simulink model "FSI07"  (R2024b)
settings: Solver=VariableStepAuto  StartTime=0.0  StopTime=t_stop  FixedStep=0.001  MaxStep=0.001  RelTol=1e-3
values from neighbouring files (symbols this model uses):
  cphi = 0.1    [FSI05WS.m]    (also in FSI06WS.m; FSI07WS.m)
  I0 = 0    [FSI03WS.m]    (also in FSI05WS.m = 0.0001; FSI06WS.m = 0.0001; FSI07WS.m = 0.0001)
  I_regulator_D = 0    [FSI07WS.m]
  I_regulator_I = 100000    [FSI07WS.m]
  I_regulator_N = 0    [FSI07WS.m]
  I_regulator_P = 1000    [FSI07WS.m]
  I_zadana = 0    [FSI07WS.m]
  integrator = 10    [FSI07WS.m]
  L = 0.02    [FSI03WS.m]    (also in FSI05WS.m = 0.05; FSI06WS.m = 0.05; FSI07WS.m = 0.05; FSI10WS.m = 0.3)
  M = 0    [FSI05WS.m]    (also in FSI06WS.m = 0.2; FSI07WS.m = 0.04; FSI10WS.m = 3)
  omega_zadana = 100    [FSI06WS.m]    (also in FSI07WS.m)
  R = 5    [FSI03WS.m]    (also in FSI05WS.m = 0; FSI06WS.m = 20; FSI07WS.m = 20)
  saturator = 0.5    [FSI07WS.m]
  step_t = 2    [FSI05WS.m]    (also in FSI06WS.m = 1; FSI07WS.m = 0.5)
  w_regulator_D = 0    [FSI07WS.m]
  w_regulator_I = 100    [FSI07WS.m]
  w_regulator_N = 0    [FSI07WS.m]
  w_regulator_P = 4    [FSI07WS.m]
libraries: slpidlib x4
settings Model: Creator=fmiro  LastModifiedBy=fmiro

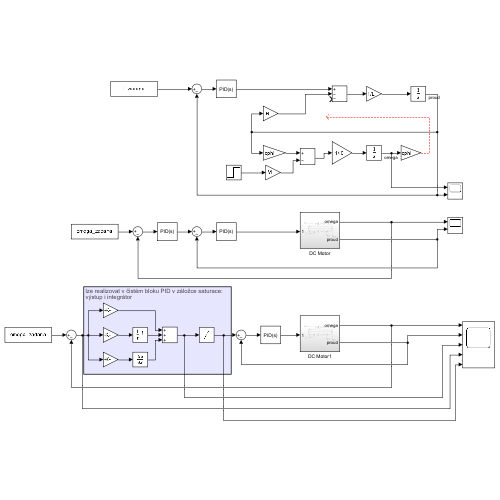
[thumbnail: Simulink's stored preview of the top-level diagram]
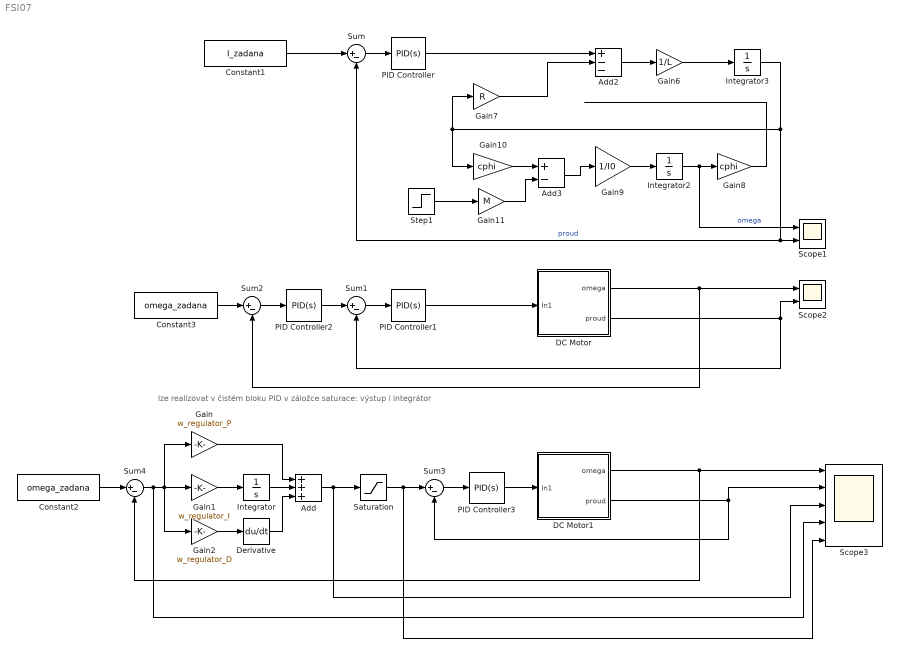
== system FSI07 ==
  note: lze realizovat v čistém bloku PID v záložce saturace:
      | výstup i integrátor
  Add : Sum  Inputs=+++
  Add2 : Sum  Inputs=+--
  Add3 : Sum  Inputs=+-
  Constant1 : Constant  Value=I_zadana
  Constant2 : Constant  Value=omega_zadana
  Constant3 : Constant  Value=omega_zadana
  DC Motor : Subsystem
  DC Motor1 : Subsystem
  Derivative : Derivative
  Gain : Gain  Gain=w_regulator_P
  Gain1 : Gain  Gain=w_regulator_I
  Gain10 : Gain  Gain=cphi
  Gain11 : Gain  Gain=M
  Gain2 : Gain  Gain=w_regulator_D
  Gain6 : Gain  Gain=1/L
  Gain7 : Gain  Gain=R
  Gain8 : Gain  Gain=cphi
  Gain9 : Gain  Gain=1/I0
  Integrator : Integrator  LimitOutput=on  UpperSaturationLimit=integrator  LowerSaturationLimit=-integrator
  Integrator2 : Integrator
  Integrator3 : Integrator
  PID Controller : slpidlib/PID Controller  Controller=PID  Form=Parallel  TimeDomain=Continuous-time  UseExternalTs=off  SampleTime=-1  IntegratorMethod=Forward Euler  FilterMethod=Forward Euler  ControllerParametersSource=internal  P=I_regulator_P  I=I_regulator_I  UseKiTs=off  D=I_regulator_D  UseExternalDerivativeSource=off  N=I_regulator_N  UseFilter=on  TunerSelectOption=Transfer Function Based (PID Tuner App)  InitialConditionSource=internal  InitialConditionForIntegrator=0  InitialConditionForFilter=0  DifferentiatorICPrevScaledInput=0  ExternalReset=none  TrackingMode=off  Kt=1  LimitOutput=off  SatLimitsSource=internal  UpperSaturationLimit=inf  LowerSaturationLimit=-inf  LinearizeAsGain=on  AntiWindupMode=none  Kb=1  LimitIntegrator=off  UpperIntegratorSaturationLimit=inf  LowerIntegratorSaturationLimit=-inf  POutMin=[]  POutMax=[]  IOutMin=[]  IOutMax=[]  DOutMin=[]  DOutMax=[]  NOutMin=[]  NOutMax=[]  SumOutMin=[]  SumOutMax=[]  SaturationOutMin=[]  SaturationOutMax=[]  PParamMin=[]  PParamMax=[]  IParamMin=[]  IParamMax=[]  DParamMin=[]  DParamMax=[]  NParamMin=[]  NParamMax=[]  KbParamMin=[]  KbParamMax=[]  KtParamMin=[]  KtParamMax=[]  KbOutMin=[]  KbOutMax=[]  KtOutMin=[]  KtOutMax=[]  IntegratorOutMin=[]  IntegratorOutMax=[]  FilterOutMin=[]  FilterOutMax=[]  SumI1OutMin=[]  SumI1OutMax=[]  SumI2OutMin=[]  SumI2OutMax=[]  SumI3OutMin=[]  SumI3OutMax=[]  SumI4OutMin=[]  SumI4OutMax=[]  SumDOutMin=[]  SumDOutMax=[]  DifferentiatorOutMin=[]  DifferentiatorOutMax=[]  FilterDiffOutCoefMin=[]  FilterDiffOutCoefMax=[]  ReciprocalOutMin=[]  ReciprocalOutMax=[]  SumDenOutMin=[]  SumDenOutMax=[]  SumNumOutMin=[]  SumNumOutMax=[]  DivideOutMin=[]  DivideOutMax=[]  UdiffTsProdOutMin=[]  UdiffTsProdOutMax=[]  NTsProdOutMin=[]  NTsProdOutMax=[]  UintegralTsProdOutMin=[]  UintegralTsProdOutMax=[]  UngainTsProdOutMin=[]  UngainTsProdOutMax=[]  ClampingZeroOutDataTypeStr=Inherit: Inherit via back propagation  ClampingZeroOutMin=[]  ClampingZeroOutMax=[]  FilterDenConstantOutDataTypeStr=Inherit: Inherit via back propagation  FilterDenConstantOutMin=[]  FilterDenConstantOutMax=[]  PCopyOutDataTypeStr=Inherit: Inherit via back propagation  PCopyOutMin=[]  PCopyOutMax=[]  NCopyOutDataTypeStr=Inherit: Inherit via back propagation  NCopyOutMin=[]  NCopyOutMax=[]  IntegratorContinuousStateAttributes=''  IntegratorStateMustResolveToSignalObject=off  IntegratorRTWStateStorageClass=Auto  FilterContinuousStateAttributes=''  FilterStateMustResolveToSignalObject=off  FilterRTWStateStorageClass=Auto  ParallelPVariant=InternalParameters  IdealPVariant=Disabled  IVariant=InternalParameters  DVariant=InternalParameters  IntegratorVariant=Continuous  SatVariant=Disabled  AWVariant=Passthrough  PCopyVariant=Disabled  TRVariant=Disabled  FdbkBlocksVariant=Forward  IdealPFdbkVariant=Disabled  SatFdbkVariant=Disabled  DerivativeFilterVariant=ContFilter  NVariant=InternalParameters  NCopyVariant=Disabled  FilterICVariant=InternalICsFilter  IntegratorICVariant=InternalICs  ExternalResetVariant=Disabled  TRSumVariant=Passthrough  SumFdbkVariant=Disabled  SumVariant=Sum_PID  TsampFilterVariant=InternalTs  TsampNgainVariant=Passthrough  TsampIntegralVariant=Disabled_SignalSpec  ExternalSaturationOutDataTypeStr=Inherit: Same as second input  DerivativeSourceVariant=ErrorSignal  PreIntVariant=InternalPreInt
  PID Controller1 : slpidlib/PID Controller  Controller=PID  Form=Parallel  TimeDomain=Continuous-time  UseExternalTs=off  SampleTime=-1  IntegratorMethod=Forward Euler  FilterMethod=Forward Euler  ControllerParametersSource=internal  P=I_regulator_P  I=I_regulator_I  UseKiTs=off  D=I_regulator_D  UseExternalDerivativeSource=off  N=I_regulator_N  UseFilter=on  TunerSelectOption=Transfer Function Based (PID Tuner App)  InitialConditionSource=internal  InitialConditionForIntegrator=0  InitialConditionForFilter=0  DifferentiatorICPrevScaledInput=0  ExternalReset=none  TrackingMode=off  Kt=1  LimitOutput=off  SatLimitsSource=internal  UpperSaturationLimit=inf  LowerSaturationLimit=-inf  LinearizeAsGain=on  AntiWindupMode=none  Kb=1  LimitIntegrator=off  UpperIntegratorSaturationLimit=inf  LowerIntegratorSaturationLimit=-inf  POutMin=[]  POutMax=[]  IOutMin=[]  IOutMax=[]  DOutMin=[]  DOutMax=[]  NOutMin=[]  NOutMax=[]  SumOutMin=[]  SumOutMax=[]  SaturationOutMin=[]  SaturationOutMax=[]  PParamMin=[]  PParamMax=[]  IParamMin=[]  IParamMax=[]  DParamMin=[]  DParamMax=[]  NParamMin=[]  NParamMax=[]  KbParamMin=[]  KbParamMax=[]  KtParamMin=[]  KtParamMax=[]  KbOutMin=[]  KbOutMax=[]  KtOutMin=[]  KtOutMax=[]  IntegratorOutMin=[]  IntegratorOutMax=[]  FilterOutMin=[]  FilterOutMax=[]  SumI1OutMin=[]  SumI1OutMax=[]  SumI2OutMin=[]  SumI2OutMax=[]  SumI3OutMin=[]  SumI3OutMax=[]  SumI4OutMin=[]  SumI4OutMax=[]  SumDOutMin=[]  SumDOutMax=[]  DifferentiatorOutMin=[]  DifferentiatorOutMax=[]  FilterDiffOutCoefMin=[]  FilterDiffOutCoefMax=[]  ReciprocalOutMin=[]  ReciprocalOutMax=[]  SumDenOutMin=[]  SumDenOutMax=[]  SumNumOutMin=[]  SumNumOutMax=[]  DivideOutMin=[]  DivideOutMax=[]  UdiffTsProdOutMin=[]  UdiffTsProdOutMax=[]  NTsProdOutMin=[]  NTsProdOutMax=[]  UintegralTsProdOutMin=[]  UintegralTsProdOutMax=[]  UngainTsProdOutMin=[]  UngainTsProdOutMax=[]  ClampingZeroOutDataTypeStr=Inherit: Inherit via back propagation  ClampingZeroOutMin=[]  ClampingZeroOutMax=[]  FilterDenConstantOutDataTypeStr=Inherit: Inherit via back propagation  FilterDenConstantOutMin=[]  FilterDenConstantOutMax=[]  PCopyOutDataTypeStr=Inherit: Inherit via back propagation  PCopyOutMin=[]  PCopyOutMax=[]  NCopyOutDataTypeStr=Inherit: Inherit via back propagation  NCopyOutMin=[]  NCopyOutMax=[]  IntegratorContinuousStateAttributes=''  IntegratorStateMustResolveToSignalObject=off  IntegratorRTWStateStorageClass=Auto  FilterContinuousStateAttributes=''  FilterStateMustResolveToSignalObject=off  FilterRTWStateStorageClass=Auto  ParallelPVariant=InternalParameters  IdealPVariant=Disabled  IVariant=InternalParameters  DVariant=InternalParameters  IntegratorVariant=Continuous  SatVariant=Disabled  AWVariant=Passthrough  PCopyVariant=Disabled  TRVariant=Disabled  FdbkBlocksVariant=Forward  IdealPFdbkVariant=Disabled  SatFdbkVariant=Disabled  DerivativeFilterVariant=ContFilter  NVariant=InternalParameters  NCopyVariant=Disabled  FilterICVariant=InternalICsFilter  IntegratorICVariant=InternalICs  ExternalResetVariant=Disabled  TRSumVariant=Passthrough  SumFdbkVariant=Disabled  SumVariant=Sum_PID  TsampFilterVariant=InternalTs  TsampNgainVariant=Passthrough  TsampIntegralVariant=Disabled_SignalSpec  ExternalSaturationOutDataTypeStr=Inherit: Same as second input  DerivativeSourceVariant=ErrorSignal  PreIntVariant=InternalPreInt
  PID Controller2 : slpidlib/PID Controller  Controller=PID  Form=Parallel  TimeDomain=Continuous-time  UseExternalTs=off  SampleTime=-1  IntegratorMethod=Forward Euler  FilterMethod=Forward Euler  ControllerParametersSource=internal  P=w_regulator_P  I=w_regulator_I  UseKiTs=off  D=w_regulator_D  UseExternalDerivativeSource=off  N=w_regulator_N  UseFilter=on  TunerSelectOption=Transfer Function Based (PID Tuner App)  InitialConditionSource=internal  InitialConditionForIntegrator=0  InitialConditionForFilter=0  DifferentiatorICPrevScaledInput=0  ExternalReset=none  TrackingMode=off  Kt=1  LimitOutput=off  SatLimitsSource=internal  UpperSaturationLimit=inf  LowerSaturationLimit=-inf  LinearizeAsGain=on  AntiWindupMode=none  Kb=1  LimitIntegrator=off  UpperIntegratorSaturationLimit=inf  LowerIntegratorSaturationLimit=-inf  POutMin=[]  POutMax=[]  IOutMin=[]  IOutMax=[]  DOutMin=[]  DOutMax=[]  NOutMin=[]  NOutMax=[]  SumOutMin=[]  SumOutMax=[]  SaturationOutMin=[]  SaturationOutMax=[]  PParamMin=[]  PParamMax=[]  IParamMin=[]  IParamMax=[]  DParamMin=[]  DParamMax=[]  NParamMin=[]  NParamMax=[]  KbParamMin=[]  KbParamMax=[]  KtParamMin=[]  KtParamMax=[]  KbOutMin=[]  KbOutMax=[]  KtOutMin=[]  KtOutMax=[]  IntegratorOutMin=[]  IntegratorOutMax=[]  FilterOutMin=[]  FilterOutMax=[]  SumI1OutMin=[]  SumI1OutMax=[]  SumI2OutMin=[]  SumI2OutMax=[]  SumI3OutMin=[]  SumI3OutMax=[]  SumI4OutMin=[]  SumI4OutMax=[]  SumDOutMin=[]  SumDOutMax=[]  DifferentiatorOutMin=[]  DifferentiatorOutMax=[]  FilterDiffOutCoefMin=[]  FilterDiffOutCoefMax=[]  ReciprocalOutMin=[]  ReciprocalOutMax=[]  SumDenOutMin=[]  SumDenOutMax=[]  SumNumOutMin=[]  SumNumOutMax=[]  DivideOutMin=[]  DivideOutMax=[]  UdiffTsProdOutMin=[]  UdiffTsProdOutMax=[]  NTsProdOutMin=[]  NTsProdOutMax=[]  UintegralTsProdOutMin=[]  UintegralTsProdOutMax=[]  UngainTsProdOutMin=[]  UngainTsProdOutMax=[]  ClampingZeroOutDataTypeStr=Inherit: Inherit via back propagation  ClampingZeroOutMin=[]  ClampingZeroOutMax=[]  FilterDenConstantOutDataTypeStr=Inherit: Inherit via back propagation  FilterDenConstantOutMin=[]  FilterDenConstantOutMax=[]  PCopyOutDataTypeStr=Inherit: Inherit via back propagation  PCopyOutMin=[]  PCopyOutMax=[]  NCopyOutDataTypeStr=Inherit: Inherit via back propagation  NCopyOutMin=[]  NCopyOutMax=[]  IntegratorContinuousStateAttributes=''  IntegratorStateMustResolveToSignalObject=off  IntegratorRTWStateStorageClass=Auto  FilterContinuousStateAttributes=''  FilterStateMustResolveToSignalObject=off  FilterRTWStateStorageClass=Auto  ParallelPVariant=InternalParameters  IdealPVariant=Disabled  IVariant=InternalParameters  DVariant=InternalParameters  IntegratorVariant=Continuous  SatVariant=Disabled  AWVariant=Passthrough  PCopyVariant=Disabled  TRVariant=Disabled  FdbkBlocksVariant=Forward  IdealPFdbkVariant=Disabled  SatFdbkVariant=Disabled  DerivativeFilterVariant=ContFilter  NVariant=InternalParameters  NCopyVariant=Disabled  FilterICVariant=InternalICsFilter  IntegratorICVariant=InternalICs  ExternalResetVariant=Disabled  TRSumVariant=Passthrough  SumFdbkVariant=Disabled  SumVariant=Sum_PID  TsampFilterVariant=InternalTs  TsampNgainVariant=Passthrough  TsampIntegralVariant=Disabled_SignalSpec  ExternalSaturationOutDataTypeStr=Inherit: Same as second input  DerivativeSourceVariant=ErrorSignal  PreIntVariant=InternalPreInt
  PID Controller3 : slpidlib/PID Controller  Controller=PID  Form=Parallel  TimeDomain=Continuous-time  UseExternalTs=off  SampleTime=-1  IntegratorMethod=Forward Euler  FilterMethod=Forward Euler  ControllerParametersSource=internal  P=I_regulator_P  I=I_regulator_I  UseKiTs=off  D=I_regulator_D  UseExternalDerivativeSource=off  N=I_regulator_N  UseFilter=on  TunerSelectOption=Transfer Function Based (PID Tuner App)  InitialConditionSource=internal  InitialConditionForIntegrator=0  InitialConditionForFilter=0  DifferentiatorICPrevScaledInput=0  ExternalReset=none  TrackingMode=off  Kt=1  LimitOutput=off  SatLimitsSource=internal  UpperSaturationLimit=inf  LowerSaturationLimit=-inf  LinearizeAsGain=on  AntiWindupMode=none  Kb=1  LimitIntegrator=off  UpperIntegratorSaturationLimit=inf  LowerIntegratorSaturationLimit=-inf  POutMin=[]  POutMax=[]  IOutMin=[]  IOutMax=[]  DOutMin=[]  DOutMax=[]  NOutMin=[]  NOutMax=[]  SumOutMin=[]  SumOutMax=[]  SaturationOutMin=[]  SaturationOutMax=[]  PParamMin=[]  PParamMax=[]  IParamMin=[]  IParamMax=[]  DParamMin=[]  DParamMax=[]  NParamMin=[]  NParamMax=[]  KbParamMin=[]  KbParamMax=[]  KtParamMin=[]  KtParamMax=[]  KbOutMin=[]  KbOutMax=[]  KtOutMin=[]  KtOutMax=[]  IntegratorOutMin=[]  IntegratorOutMax=[]  FilterOutMin=[]  FilterOutMax=[]  SumI1OutMin=[]  SumI1OutMax=[]  SumI2OutMin=[]  SumI2OutMax=[]  SumI3OutMin=[]  SumI3OutMax=[]  SumI4OutMin=[]  SumI4OutMax=[]  SumDOutMin=[]  SumDOutMax=[]  DifferentiatorOutMin=[]  DifferentiatorOutMax=[]  FilterDiffOutCoefMin=[]  FilterDiffOutCoefMax=[]  ReciprocalOutMin=[]  ReciprocalOutMax=[]  SumDenOutMin=[]  SumDenOutMax=[]  SumNumOutMin=[]  SumNumOutMax=[]  DivideOutMin=[]  DivideOutMax=[]  UdiffTsProdOutMin=[]  UdiffTsProdOutMax=[]  NTsProdOutMin=[]  NTsProdOutMax=[]  UintegralTsProdOutMin=[]  UintegralTsProdOutMax=[]  UngainTsProdOutMin=[]  UngainTsProdOutMax=[]  ClampingZeroOutDataTypeStr=Inherit: Inherit via back propagation  ClampingZeroOutMin=[]  ClampingZeroOutMax=[]  FilterDenConstantOutDataTypeStr=Inherit: Inherit via back propagation  FilterDenConstantOutMin=[]  FilterDenConstantOutMax=[]  PCopyOutDataTypeStr=Inherit: Inherit via back propagation  PCopyOutMin=[]  PCopyOutMax=[]  NCopyOutDataTypeStr=Inherit: Inherit via back propagation  NCopyOutMin=[]  NCopyOutMax=[]  IntegratorContinuousStateAttributes=''  IntegratorStateMustResolveToSignalObject=off  IntegratorRTWStateStorageClass=Auto  FilterContinuousStateAttributes=''  FilterStateMustResolveToSignalObject=off  FilterRTWStateStorageClass=Auto  ParallelPVariant=InternalParameters  IdealPVariant=Disabled  IVariant=InternalParameters  DVariant=InternalParameters  IntegratorVariant=Continuous  SatVariant=Disabled  AWVariant=Passthrough  PCopyVariant=Disabled  TRVariant=Disabled  FdbkBlocksVariant=Forward  IdealPFdbkVariant=Disabled  SatFdbkVariant=Disabled  DerivativeFilterVariant=ContFilter  NVariant=InternalParameters  NCopyVariant=Disabled  FilterICVariant=InternalICsFilter  IntegratorICVariant=InternalICs  ExternalResetVariant=Disabled  TRSumVariant=Passthrough  SumFdbkVariant=Disabled  SumVariant=Sum_PID  TsampFilterVariant=InternalTs  TsampNgainVariant=Passthrough  TsampIntegralVariant=Disabled_SignalSpec  ExternalSaturationOutDataTypeStr=Inherit: Same as second input  DerivativeSourceVariant=ErrorSignal  PreIntVariant=InternalPreInt
  Saturation : Saturate  UpperLimit=saturator  LowerLimit=-saturator
  Scope1 : Scope  NumInputPorts=2
  Scope2 : Scope  NumInputPorts=2
  Scope3 : Scope  NumInputPorts=5
  Step1 : Step  Time=step_t  SampleTime=0
  Sum{,1..4} (5 alike) : Sum  Inputs=|+-
  wires:
  Integrator2/1 -> Scope1/1, Gain8/1  "omega"
  Add3/1 -> Gain9/1
  Gain7/1 -> Add2/2
  Gain9/1 -> Integrator2/1
  Step1/1 -> Gain11/1
  Gain11/1 -> Add3/2
  Gain10/1 -> Add3/1
  Add2/1 -> Gain6/1
  Gain6/1 -> Integrator3/1
  Integrator3/1 -> Sum/2, Scope1/2, Gain10/1, Gain7/1  "proud"
  PID Controller/1 -> Add2/1
  Sum/1 -> PID Controller/1
  Constant1/1 -> Sum/1
  Gain8/1 -> ?
  Sum1/1 -> PID Controller1/1
  PID Controller2/1 -> Sum1/1
  Sum2/1 -> PID Controller2/1
  Constant3/1 -> Sum2/1
  DC Motor/1(omega) -> Sum2/2, Scope2/1
  DC Motor/2(proud) -> Sum1/2, Scope2/2
  PID Controller1/1 -> DC Motor/1(In1)
  DC Motor1/2(proud) -> Scope3/2, Sum3/2
  DC Motor1/1(omega) -> Sum4/2, Scope3/1
  PID Controller3/1 -> DC Motor1/1(In1)
  Sum3/1 -> PID Controller3/1
  Constant2/1 -> Sum4/1
  Add/1 -> Scope3/3, Saturation/1
  Integrator/1 -> Add/2
  Gain/1 -> Add/1
  Gain2/1 -> Derivative/1
  Gain1/1 -> Integrator/1
  Sum4/1 -> Scope3/4, Gain/1, Gain2/1, Gain1/1
  Saturation/1 -> Scope3/5, Sum3/1
  Derivative/1 -> Add/3

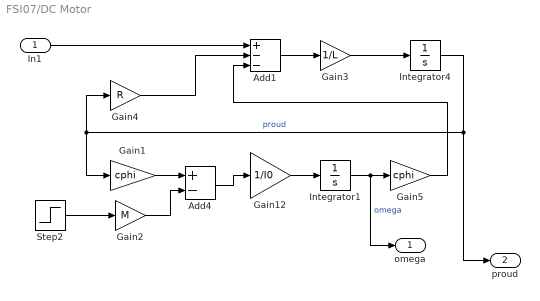
== system FSI07/DC Motor ==
  In1 : Inport
  Add1 : Sum  Inputs=+--
  Add4 : Sum  Inputs=+-
  Gain1 : Gain  Gain=cphi
  Gain12 : Gain  Gain=1/I0
  Gain2 : Gain  Gain=M
  Gain3 : Gain  Gain=1/L
  Gain4 : Gain  Gain=R
  Gain5 : Gain  Gain=cphi
  Integrator1 : Integrator
  Integrator4 : Integrator
  Step2 : Step  Time=step_t  SampleTime=0
  omega : Outport
  proud : Outport  Port=2
  wires:
  Integrator4/1 -> proud/1, Gain1/1, Gain4/1  "proud"
  Gain1/1 -> Add4/1
  Integrator1/1 -> omega/1, Gain5/1  "omega"
  Gain12/1 -> Integrator1/1
  Gain2/1 -> Add4/2
  Add4/1 -> Gain12/1
  Gain3/1 -> Integrator4/1
  Step2/1 -> Gain2/1
  Add1/1 -> Gain3/1
  Gain4/1 -> Add1/2
  Gain5/1 -> Add1/3
  In1/1 -> Add1/1

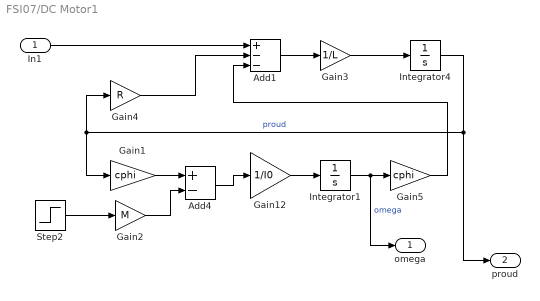
== system FSI07/DC Motor1 ==
  In1 : Inport
  Add1 : Sum  Inputs=+--
  Add4 : Sum  Inputs=+-
  Gain1 : Gain  Gain=cphi
  Gain12 : Gain  Gain=1/I0
  Gain2 : Gain  Gain=M
  Gain3 : Gain  Gain=1/L
  Gain4 : Gain  Gain=R
  Gain5 : Gain  Gain=cphi
  Integrator1 : Integrator
  Integrator4 : Integrator
  Step2 : Step  Time=step_t  SampleTime=0
  omega : Outport
  proud : Outport  Port=2
  wires:
  Integrator4/1 -> proud/1, Gain1/1, Gain4/1  "proud"
  Gain1/1 -> Add4/1
  Integrator1/1 -> omega/1, Gain5/1  "omega"
  Gain12/1 -> Integrator1/1
  Gain2/1 -> Add4/2
  Add4/1 -> Gain12/1
  Gain3/1 -> Integrator4/1
  Step2/1 -> Gain2/1
  Add1/1 -> Gain3/1
  Gain4/1 -> Add1/2
  Gain5/1 -> Add1/3
  In1/1 -> Add1/1
